simulink model "hdlFrame_homography"  (R2024a)
settings: Solver=FixedStepDiscrete  StartTime=0.0  StopTime=10.0  RelTol=1e-3
undefined symbols (not defined in the file or in its folder): gray
settings Model: DataTypeOverride=Off  Creator=navan  LastModifiedBy=navan
settings OptimizationCC: BlockReduction=off  ConditionallyExecuteInputs=off  DefaultParameterBehavior=Inlined  InheritOutputTypeSmallerThanSingle=on
settings DebuggingCC: AlgebraicLoopMsg=error  SingleTaskRateTransMsg=error
settings HardwareCC: ProdBitPerPointer=32  ProdBitPerSizeT=32  ProdBitPerPtrDiffT=32  ProdLargestAtomicFloat=None  ProdIntDivRoundTo=Undefined  ProdEndianess=Unspecified  ProdWordSize=32  ProdHWDeviceType=ASIC/FPGA->ASIC/FPGA  TargetBitPerPointer=64  TargetBitPerSizeT=64  TargetBitPerPtrDiffT=64  TargetLongLongMode=on  TargetIntDivRoundTo=Zero  TargetEndianess=LittleEndian  TargetWordSize=64  TargetHWDeviceType=Custom Processor->MATLAB Host Computer  ProdEqTarget=off

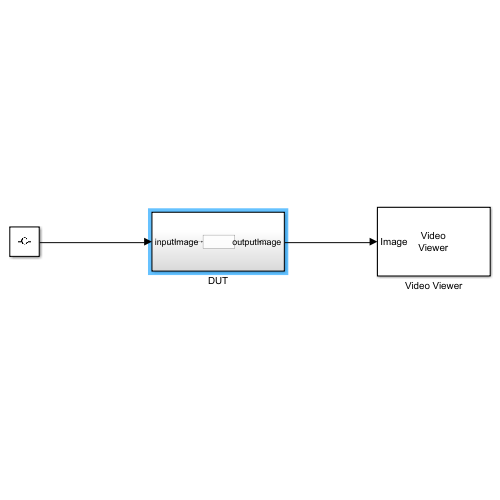
[thumbnail: Simulink's stored preview of the top-level diagram]
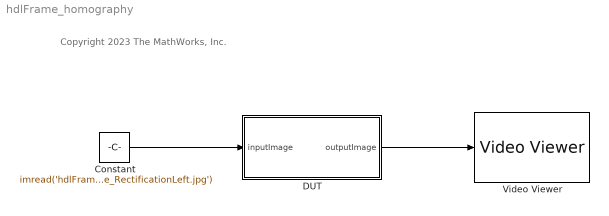
== system hdlFrame_homography ==
  note: Copyright 2023 The MathWorks, Inc.
  Constant : Constant  Value=imread('hdlFrame_RectificationLeft.jpg')  VectorParams1D=off  SampleTime=1
  DUT : Subsystem
  Video Viewer : VideoViewer  colormapValue=gray(256)  FigPos=[105 794 470 421.333333333333]
  wires:
  Constant/1 -> DUT/1(inputImage)
  DUT/1(outputImage) -> Video Viewer/1

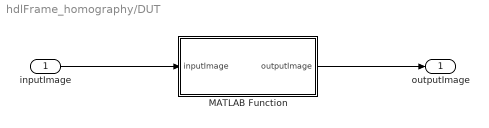
== system hdlFrame_homography/DUT ==
  inputImage : Inport
  MATLAB Function : MATLAB Function  TreatAsAtomicUnit=on
  outputImage : Outport
  wires:
  MATLAB Function/1(outputImage) -> outputImage/1
  inputImage/1 -> MATLAB Function/1(inputImage)

== matlab function hdlFrame_homography/DUT/MATLAB Function ==
  data: inputImage input; outputImage output
function outputImage  = rectifyOneImage(inputImage)
H = coder.load('hdlFrame_homography.mat');
rows = 480;
cols = 752;
MAX_OFFSET = 12;
neighborhood_size = [MAX_OFFSET*2-1 MAX_OFFSET*2-1];

outputImage = hdl.npufun(@doMapping, neighborhood_size, inputImage, 'KernelArg', H.leftH, ...
    'KernelArg', rows, 'KernelArg', cols, 'KernelArg', MAX_OFFSET, ...
    'BoundaryMethod', 'replicate');
end

function output = doMapping(input, leftH, height, width, offset)

persistent row col
if isempty(row)
    row = uint32(1);
    col = uint32(1);
end

vector = [col;row;1];
result = leftH' * single(vector);
result = result./result(3);

% note that for now these are rounded to whole pixels
% future state would keep fractional pixels for interpolation stage
xMapping = round(result(1));
yMapping = round(result(2));

% only map to indices that are in the original unrectified image
if xMapping < 1
    xMapping = single(1);
end
if xMapping > width
    xMapping = single(width);
end
if yMapping < 1
    yMapping = single(1);
end
if yMapping > height
    yMapping = single(height);
end

% Find offset into neighborhood
xMapping = xMapping - single(col) + offset;
yMapping = yMapping - single(row) + offset;

% set intensity values of rectified image
output = input(yMapping,xMapping);

% update row and col counters
% Update the row/column trackers
if row == height && col == width
    row = uint32(1);
    col = uint32(1);
elseif col == width
    row = row + 1;
    col = uint32(1);
else
    col = col + 1;
end

end
